simulink model "dec_fir_dbl_col_test"  (Simulink 7.2)
settings: Solver=FixedStepDiscrete  SolverMode=SingleTasking  StartTime=0.0  StopTime=50  RelTol=1e-3
libraries: xbsIndex_r4 x50, casper_library_downconverter x8, casper_library_misc x2
settings Model: Creator=User  LastModifiedBy=root
settings OptimizationCC: InitFltsAndDblsToZero=on

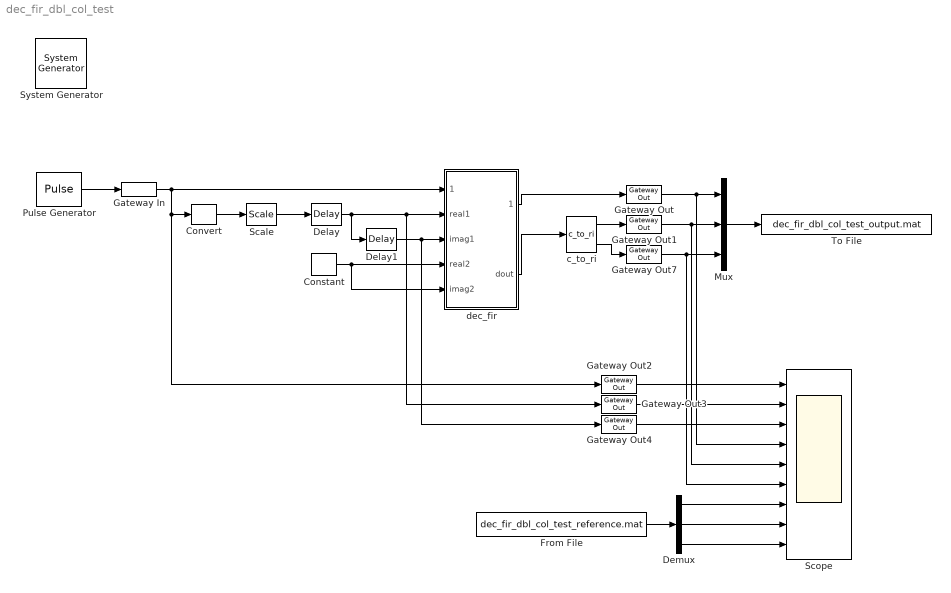
== system dec_fir_dbl_col_test ==
  " System Generator" : xbsIndex_r4/ System Generator  Tag=genX  SystemSampleTime=-1  xilinxfamily=Virtex4  part=xc4vsx35  speed=-10  package=ff668  synthesis_tool=XST  clock_wrapper=Clock Enables  directory=./netlist  testbench=off  simulink_period=1  sysclk_period=100  dcm_input_clock_period=100  incr_netlist=off  trim_vbits=Everywhere in SubSystem  dbl_ovrd=According to Block Masks  core_generation=According to Block Masks  run_coregen=off  deprecated_control=off  eval_field=0  block_type=sysgen
      settings: block_version=10.1.1
  Constant : xbsIndex_r4/Constant  arith_type=Signed (2's comp)  const=0  n_bits=10  bin_pt=9  explicit_period=on  period=1  equ=P=C  opselect=C  inp2=PCIN>>17  opr=+  inp1=P  carry=CIN  dbl_ovrd=off  block_type=constant
      settings: block_version=11.4
  Convert : xbsIndex_r4/Convert  arith_type="Signed  (2's comp)"  n_bits=10  bin_pt=8  quantization=Truncate  overflow=Wrap  latency=0  dbl_ovrd=off  pipeline=off  block_type=convert
      settings: block_version=11.4
  Delay : xbsIndex_r4/Delay  en=off  latency=1  dbl_ovrd=off  reg_retiming=off  block_type=delay
      settings: block_version=11.4
  Delay1 : xbsIndex_r4/Delay  en=off  latency=1  dbl_ovrd=off  reg_retiming=off  block_type=delay
      settings: block_version=11.4
  Demux : Demux  Outputs=3
  From File : FromFile  FileName=dec_fir_dbl_col_test_reference.mat  SampleTime=1
  Gateway In : xbsIndex_r4/Gateway In  arith_type=Boolean  n_bits=16  bin_pt=14  quantization="Round  (unbiased: +/- Inf)"  overflow=Saturate  period=1  dbl_ovrd=off  timing_constraint=None  locs_specified=off  LOCs={}  hdl_port=on  block_type=gatewayin
      settings: infoedit="Gateway in block.  Converts inputs of type Simulink integer, double and fixed point to  Xilinx fixed point type.<P><P>Hardware notes:  In hardware these blocks become top level input ports."  block_version=10.1.1
  Gateway Out{,1..4,7} (6 alike) : xbsIndex_r4/Gateway Out  hdl_port=on  timing_constraint=None  locs_specified=off  LOCs={}  block_type=gatewayout
      settings: infoedit="Gateway out block.  Converts Xilinx fixed point inputs into ouputs of type Simulink integer, double, or fixed point.<br><br>Hardware notes:  In hardware these blocks become top level output ports or are discarded, depending on how they are configured."  block_version=11.4
  Mux : Mux  Inputs=3
  Pulse Generator : DiscretePulseGenerator  Period=128  PhaseDelay=15
  Scale : xbsIndex_r4/Scale  scale_factor=-1  dbl_ovrd=off  block_type=scale
  Scope : Scope  NumInputPorts=9
      settings: YMin=-5~-5~-5~-5~-5~-5~-5~-5~-5  YMax=5~5~5~5~5~5~5~5~5
  To File : ToFile  Filename=dec_fir_dbl_col_test_output.mat  MatrixName=output
  c_to_ri : casper_library_misc/c_to_ri  SystemSampleTime=-1  n_bits=10  bin_pt=9
      settings: AttributesFormatString=10_9 r/i
  dec_fir : Subsystem  AncestorBlock=casper_library_downconverter/dec_fir  mask(dec_fir){n_inputs=2, coeff=getfield( getfield( get_param( gcb,'UserData' ), 'parameters'),'coeff'), n_bits=10, quantization=Round  (unbiased: Even Values), add_latency=2, mult_latency=3, conv_latency=2, coeff_bit_width=18, coeff_bin_pt=17, absorb_adders=off, adder_imp=DSP48}
      mask prompts: n_inputs "Number of Parallel Streams"; coeff "Coefficients"; n_bits "Bit Width Out"; quantization "Quantization Behavior"; add_latency "Add Latency"; mult_latency "Mult Latency"; conv_latency "Convert latency"; coeff_bit_width "Coefficient bit width"; coeff_bin_pt "Coefficient binary point"; absorb_adders "Absorb adders into DSP slices"; adder_imp "Adder implementation"
      mask help: FIR filter which can handle multiple time samples in parallel and decimates down to 1 time sample. If coefficients are symmetric, will automatically fold before multiplying.
      mask init:
      | dec_fir_init(gcb, ...
      |     'n_inputs', n_inputs, ...
      |     'coeff', coeff, ...
      |     'n_bits', n_bits, ...
      |     'quantization', quantization, ...
      |     'add_latency', add_latency, ...
      |     'mult_latency', mult_latency, ...
      |     'conv_latency', conv_latency, ...
      |     'coeff_bit_width', coeff_bit_width, ...
      |     'coeff_bin_pt', coeff_bin_pt, ...
      |     'absorb_adders', absorb_adders, ...
      |     'adder_imp', adder_imp);
      settings: AttributesFormatString=|
      | 16 taps
      | 10_9 r/i
      mask Help: eval('xlWeb(''http://casper.berkeley.edu/wiki/Dec_fir'')')
      mask StyleString: edit,edit,edit,popup(Truncate|Round  (unbiased: +/- Inf)|Round  (unbiased: Even Values)),edit,edit,edit,edit,edit,checkbox,popup(Behavioral|Fabric|DSP48)
  wires:
  Pulse Generator/1 -> Gateway In/1
  Gateway In/1 -> Convert/1, Gateway Out2/1, dec_fir/1(sync_in)
  Mux/1 -> To File/1
  Delay/1 -> Delay1/1, Gateway Out3/1, dec_fir/2(real1)
  Delay1/1 -> Gateway Out4/1, dec_fir/3(imag1)
  Convert/1 -> Scale/1
  Gateway Out/1 -> Mux/1, Scope/4
  Gateway Out2/1 -> Scope/1
  Gateway Out3/1 -> Scope/2
  Gateway Out4/1 -> Scope/3
  dec_fir/2(dout) -> c_to_ri/1
  c_to_ri/1 -> Gateway Out1/1
  c_to_ri/2 -> Gateway Out7/1
  Gateway Out1/1 -> Mux/2, Scope/5
  From File/1 -> Demux/1
  Scale/1 -> Delay/1
  dec_fir/1(sync_out) -> Gateway Out/1
  Gateway Out7/1 -> Mux/3, Scope/6
  Demux/1 -> Scope/7
  Demux/2 -> Scope/8
  Demux/3 -> Scope/9
  Constant/1 -> dec_fir/5(imag2), dec_fir/4(real2)

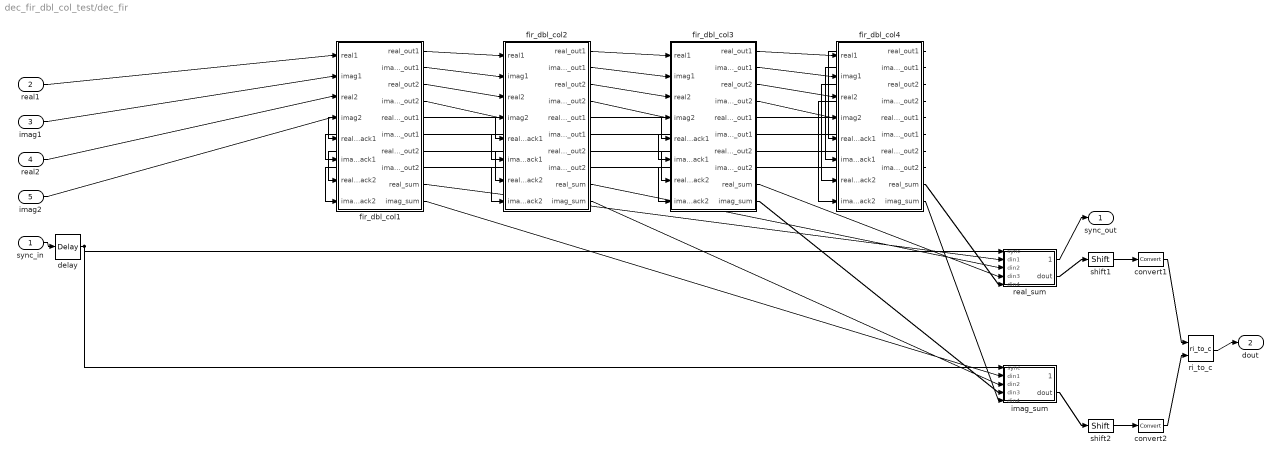
== system dec_fir_dbl_col_test/dec_fir ==
  sync_in : Inport
  real1 : Inport  Port=2
  imag1 : Inport  Port=3
  real2 : Inport  Port=4
  imag2 : Inport  Port=5
  convert1 : xbsIndex_r4/Convert  arith_type="Signed  (2's comp)"  n_bits=10  bin_pt=9  quantization="Round  (unbiased: Even Values)"  overflow=Wrap  latency=2  dbl_ovrd=off  pipeline=off  block_type=convert
      settings: block_version=11.4
  convert2 : xbsIndex_r4/Convert  arith_type="Signed  (2's comp)"  n_bits=10  bin_pt=9  quantization="Round  (unbiased: Even Values)"  overflow=Wrap  latency=2  dbl_ovrd=off  pipeline=off  block_type=convert
      settings: block_version=11.4
  delay : xbsIndex_r4/Delay  en=off  latency=9  dbl_ovrd=off  reg_retiming=off  block_type=delay
      settings: block_version=11.4
  fir_dbl_col1 : Subsystem  AncestorBlock=casper_library_downconverter/fir_dbl_col  mask(fir_dbl_col){n_inputs=2, coeff=[0.2         0.1], add_latency=2, mult_latency=3, coeff_bit_width=18, coeff_bin_pt=17, first_stage_hdl=off, adder_imp=DSP48}
      mask prompts: n_inputs "Inputs"; coeff "Coefficients"; add_latency "Add latency"; mult_latency "Mult Latency"; coeff_bit_width "Coefficient bit width"; coeff_bin_pt "Coefficient binary point"; first_stage_hdl "Implement first stage of adder trees on output as behavioural HDL"; adder_imp "Adder implementation"
      mask init:
      | fir_dbl_col_init(gcb, ...
      |     'n_inputs', n_inputs, ...
      |     'coeff', coeff, ...
      |     'mult_latency', mult_latency, ...
      |     'add_latency', add_latency, ...
      |     'coeff_bit_width', coeff_bit_width, ...
      |     'coeff_bin_pt', coeff_bin_pt,  ...
      |     'first_stage_hdl', first_stage_hdl, ...
      |     'adder_imp', adder_imp);
      mask Help: eval('xlWeb(''http://casper.berkeley.edu/wiki/Fir_dbl_col'')')
      mask StyleString: edit,edit,edit,edit,edit,edit,checkbox,popup(Behavioral|Fabric|DSP48)
  fir_dbl_col2 : Subsystem  AncestorBlock=casper_library_downconverter/fir_dbl_col  mask(fir_dbl_col){n_inputs=2, coeff=[0.4         0.3], add_latency=2, mult_latency=3, coeff_bit_width=18, coeff_bin_pt=17, first_stage_hdl=off, adder_imp=DSP48}
      mask prompts: n_inputs "Inputs"; coeff "Coefficients"; add_latency "Add latency"; mult_latency "Mult Latency"; coeff_bit_width "Coefficient bit width"; coeff_bin_pt "Coefficient binary point"; first_stage_hdl "Implement first stage of adder trees on output as behavioural HDL"; adder_imp "Adder implementation"
      mask init: same as dec_fir_dbl_col_test/dec_fir/fir_dbl_col1
      mask Help: eval('xlWeb(''http://casper.berkeley.edu/wiki/Fir_dbl_col'')')
      mask StyleString: edit,edit,edit,edit,edit,edit,checkbox,popup(Behavioral|Fabric|DSP48)
  fir_dbl_col3 : Subsystem  AncestorBlock=casper_library_downconverter/fir_dbl_col  mask(fir_dbl_col){n_inputs=2, coeff=[0.6         0.5], add_latency=2, mult_latency=3, coeff_bit_width=18, coeff_bin_pt=17, first_stage_hdl=off, adder_imp=DSP48}
      mask prompts: n_inputs "Inputs"; coeff "Coefficients"; add_latency "Add latency"; mult_latency "Mult Latency"; coeff_bit_width "Coefficient bit width"; coeff_bin_pt "Coefficient binary point"; first_stage_hdl "Implement first stage of adder trees on output as behavioural HDL"; adder_imp "Adder implementation"
      mask init: same as dec_fir_dbl_col_test/dec_fir/fir_dbl_col1
      mask Help: eval('xlWeb(''http://casper.berkeley.edu/wiki/Fir_dbl_col'')')
      mask StyleString: edit,edit,edit,edit,edit,edit,checkbox,popup(Behavioral|Fabric|DSP48)
  fir_dbl_col4 : Subsystem  AncestorBlock=casper_library_downconverter/fir_dbl_col  mask(fir_dbl_col){n_inputs=2, coeff=[0.8         0.7], add_latency=2, mult_latency=3, coeff_bit_width=18, coeff_bin_pt=17, first_stage_hdl=off, adder_imp=DSP48}
      mask prompts: n_inputs "Inputs"; coeff "Coefficients"; add_latency "Add latency"; mult_latency "Mult Latency"; coeff_bit_width "Coefficient bit width"; coeff_bin_pt "Coefficient binary point"; first_stage_hdl "Implement first stage of adder trees on output as behavioural HDL"; adder_imp "Adder implementation"
      mask init: same as dec_fir_dbl_col_test/dec_fir/fir_dbl_col1
      mask Help: eval('xlWeb(''http://casper.berkeley.edu/wiki/Fir_dbl_col'')')
      mask StyleString: edit,edit,edit,edit,edit,edit,checkbox,popup(Behavioral|Fabric|DSP48)
  imag_sum : Subsystem  AncestorBlock=casper_library_misc/adder_tree  mask(adder_tree){n_inputs=4, latency=2, adder_imp=DSP48, first_stage_hdl=off}
      mask prompts: n_inputs "Number of Inputs"; latency "Add Latency"; adder_imp "Adder implementation"; first_stage_hdl "Use behavioural HDL for first stage of adders"
      mask help:
      | Sums all inputs using a tree of adds and delays.
      |
      | Number of inputs: The number of inputs to the block to be summed
      | Add latency: The number of clock cycles to perform one addition (affects timing)..
      | Adder implementation: choice of fabric or DSP48E core, or behavioral HDL
      | Use behavioural HDL for first stage of adders: Causes the first stage of adders to be absorbed into DSP blocks if multipliers precede them (Virtex 5). Overrides Adder implementation
      mask init:
      | adder_tree_init(gcb, ...
      |     'n_inputs', n_inputs, ...
      |     'latency', latency, ...
      |     'adder_imp', adder_imp, ...
      |     'first_stage_hdl', first_stage_hdl);
      settings: AttributesFormatString=latency 4
      mask Help: eval('xlWeb(''http://casper.berkeley.edu/wiki/Adder_tree'')')
      mask StyleString: edit,edit,popup(Behavioral|Fabric|DSP48),checkbox
  real_sum : Subsystem  AncestorBlock=casper_library_misc/adder_tree  mask(adder_tree){n_inputs=4, latency=2, adder_imp=DSP48, first_stage_hdl=off}
      mask prompts: n_inputs "Number of Inputs"; latency "Add Latency"; adder_imp "Adder implementation"; first_stage_hdl "Use behavioural HDL for first stage of adders"
      mask help:
      | Sums all inputs using a tree of adds and delays.
      |
      | Number of inputs: The number of inputs to the block to be summed
      | Add latency: The number of clock cycles to perform one addition (affects timing)..
      | Adder implementation: choice of fabric or DSP48E core, or behavioral HDL
      | Use behavioural HDL for first stage of adders: Causes the first stage of adders to be absorbed into DSP blocks if multipliers precede them (Virtex 5). Overrides Adder implementation
      mask init:
      | adder_tree_init(gcb, ...
      |     'n_inputs', n_inputs, ...
      |     'latency', latency, ...
      |     'adder_imp', adder_imp, ...
      |     'first_stage_hdl', first_stage_hdl);
      settings: AttributesFormatString=latency 4
      mask Help: eval('xlWeb(''http://casper.berkeley.edu/wiki/Adder_tree'')')
      mask StyleString: edit,edit,popup(Behavioral|Fabric|DSP48),checkbox
  ri_to_c : casper_library_misc/ri_to_c  SystemSampleTime=-1
  shift1 : xbsIndex_r4/Shift  shift_dir=Left  shift_bits=1  en=off  latency=0  precision=Full  arith_type="Signed  (2's comp)"  n_bits=16  bin_pt=14  quantization=Truncate  overflow=Wrap  dbl_ovrd=off  block_type=shift
  shift2 : xbsIndex_r4/Shift  shift_dir=Left  shift_bits=1  en=off  latency=0  precision=Full  arith_type="Signed  (2's comp)"  n_bits=16  bin_pt=14  quantization=Truncate  overflow=Wrap  dbl_ovrd=off  block_type=shift
  sync_out : Outport
  dout : Outport  Port=2
  wires:
  real1/1 -> fir_dbl_col1/1(real1)
  imag1/1 -> fir_dbl_col1/2(imag1)
  real2/1 -> fir_dbl_col1/3(real2)
  imag2/1 -> fir_dbl_col1/4(imag2)
  fir_dbl_col1/9(real_sum) -> real_sum/2(din1)
  fir_dbl_col1/10(imag_sum) -> imag_sum/2(din1)
  fir_dbl_col1/1(real_out1) -> fir_dbl_col2/1(real1)
  fir_dbl_col1/2(imag_out1) -> fir_dbl_col2/2(imag1)
  fir_dbl_col1/3(real_out2) -> fir_dbl_col2/3(real2)
  fir_dbl_col1/4(imag_out2) -> fir_dbl_col2/4(imag2)
  fir_dbl_col2/9(real_sum) -> real_sum/3(din2)
  fir_dbl_col2/10(imag_sum) -> imag_sum/3(din2)
  fir_dbl_col2/1(real_out1) -> fir_dbl_col3/1(real1)
  fir_dbl_col2/2(imag_out1) -> fir_dbl_col3/2(imag1)
  fir_dbl_col2/3(real_out2) -> fir_dbl_col3/3(real2)
  fir_dbl_col2/4(imag_out2) -> fir_dbl_col3/4(imag2)
  fir_dbl_col3/9(real_sum) -> real_sum/4(din3)
  fir_dbl_col3/10(imag_sum) -> imag_sum/4(din3)
  fir_dbl_col3/1(real_out1) -> fir_dbl_col4/1(real1)
  fir_dbl_col3/2(imag_out1) -> fir_dbl_col4/2(imag1)
  fir_dbl_col3/3(real_out2) -> fir_dbl_col4/3(real2)
  fir_dbl_col3/4(imag_out2) -> fir_dbl_col4/4(imag2)
  fir_dbl_col4/9(real_sum) -> real_sum/5(din4)
  fir_dbl_col4/10(imag_sum) -> imag_sum/5(din4)
  real_sum/2(dout) -> shift1/1
  imag_sum/2(dout) -> shift2/1
  shift1/1 -> convert1/1
  shift2/1 -> convert2/1
  convert1/1 -> ri_to_c/1
  convert2/1 -> ri_to_c/2
  ri_to_c/1 -> dout/1
  sync_in/1 -> delay/1
  delay/1 -> real_sum/1(sync), imag_sum/1(sync)
  real_sum/1(sync_out) -> sync_out/1
  fir_dbl_col2/5(real_back_out1) -> fir_dbl_col1/5(real_back1)
  fir_dbl_col2/6(imag_back_out1) -> fir_dbl_col1/6(imag_back1)
  fir_dbl_col2/7(real_back_out2) -> fir_dbl_col1/7(real_back2)
  fir_dbl_col2/8(imag_back_out2) -> fir_dbl_col1/8(imag_back2)
  fir_dbl_col3/5(real_back_out1) -> fir_dbl_col2/5(real_back1)
  fir_dbl_col3/6(imag_back_out1) -> fir_dbl_col2/6(imag_back1)
  fir_dbl_col3/7(real_back_out2) -> fir_dbl_col2/7(real_back2)
  fir_dbl_col3/8(imag_back_out2) -> fir_dbl_col2/8(imag_back2)
  fir_dbl_col4/5(real_back_out1) -> fir_dbl_col3/5(real_back1)
  fir_dbl_col4/6(imag_back_out1) -> fir_dbl_col3/6(imag_back1)
  fir_dbl_col4/7(real_back_out2) -> fir_dbl_col3/7(real_back2)
  fir_dbl_col4/8(imag_back_out2) -> fir_dbl_col3/8(imag_back2)
  fir_dbl_col4/1(real_out1) -> fir_dbl_col4/5(real_back1)
  fir_dbl_col4/2(imag_out1) -> fir_dbl_col4/6(imag_back1)
  fir_dbl_col4/3(real_out2) -> fir_dbl_col4/7(real_back2)
  fir_dbl_col4/4(imag_out2) -> fir_dbl_col4/8(imag_back2)

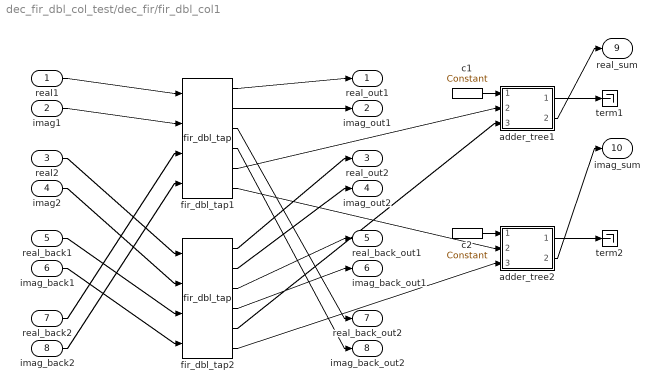
== system dec_fir_dbl_col_test/dec_fir/fir_dbl_col1 ==
  real1 : Inport
  imag1 : Inport  Port=2
  real2 : Inport  Port=3
  imag2 : Inport  Port=4
  real_back1 : Inport  Port=5
  imag_back1 : Inport  Port=6
  real_back2 : Inport  Port=7
  imag_back2 : Inport  Port=8
  adder_tree1 : Subsystem  AncestorBlock=casper_library_misc/adder_tree  mask(adder_tree){n_inputs=2, latency=2, adder_imp=DSP48, first_stage_hdl=off}
      mask prompts: n_inputs "Number of Inputs"; latency "Add Latency"; adder_imp "Adder implementation"; first_stage_hdl "Use behavioural HDL for first stage of adders"
      mask help:
      | Sums all inputs using a tree of adds and delays.
      |
      | Number of inputs: The number of inputs to the block to be summed
      | Add latency: The number of clock cycles to perform one addition (affects timing)..
      | Adder implementation: choice of fabric or DSP48E core, or behavioral HDL
      | Use behavioural HDL for first stage of adders: Causes the first stage of adders to be absorbed into DSP blocks if multipliers precede them (Virtex 5). Overrides Adder implementation
      mask init:
      | adder_tree_init(gcb, ...
      |     'n_inputs', n_inputs, ...
      |     'latency', latency, ...
      |     'adder_imp', adder_imp, ...
      |     'first_stage_hdl', first_stage_hdl);
      settings: AttributesFormatString=latency 2
      mask Help: eval('xlWeb(''http://casper.berkeley.edu/wiki/Adder_tree'')')
      mask StyleString: edit,edit,popup(Behavioral|Fabric|DSP48),checkbox
  adder_tree2 : Subsystem  AncestorBlock=casper_library_misc/adder_tree  mask(adder_tree){n_inputs=2, latency=2, adder_imp=DSP48, first_stage_hdl=off}
      mask prompts: n_inputs "Number of Inputs"; latency "Add Latency"; adder_imp "Adder implementation"; first_stage_hdl "Use behavioural HDL for first stage of adders"
      mask help:
      | Sums all inputs using a tree of adds and delays.
      |
      | Number of inputs: The number of inputs to the block to be summed
      | Add latency: The number of clock cycles to perform one addition (affects timing)..
      | Adder implementation: choice of fabric or DSP48E core, or behavioral HDL
      | Use behavioural HDL for first stage of adders: Causes the first stage of adders to be absorbed into DSP blocks if multipliers precede them (Virtex 5). Overrides Adder implementation
      mask init:
      | adder_tree_init(gcb, ...
      |     'n_inputs', n_inputs, ...
      |     'latency', latency, ...
      |     'adder_imp', adder_imp, ...
      |     'first_stage_hdl', first_stage_hdl);
      settings: AttributesFormatString=latency 2
      mask Help: eval('xlWeb(''http://casper.berkeley.edu/wiki/Adder_tree'')')
      mask StyleString: edit,edit,popup(Behavioral|Fabric|DSP48),checkbox
  c1 : xbsIndex_r4/Constant  arith_type=Signed (2's comp)  const=1  n_bits=16  bin_pt=14  explicit_period=on  period=1  equ=P=C  opselect=C  inp2=PCIN>>17  opr=+  inp1=P  carry=CIN  dbl_ovrd=off  block_type=constant
      settings: block_version=11.4
  c2 : xbsIndex_r4/Constant  arith_type=Signed (2's comp)  const=1  n_bits=16  bin_pt=14  explicit_period=on  period=1  equ=P=C  opselect=C  inp2=PCIN>>17  opr=+  inp1=P  carry=CIN  dbl_ovrd=off  block_type=constant
      settings: block_version=11.4
  fir_dbl_tap1 : casper_library_downconverter/fir_dbl_tap  SystemSampleTime=-1  factor=0.2  add_latency=2  mult_latency=3  coeff_bit_width=18  coeff_bin_pt=17
  fir_dbl_tap2 : casper_library_downconverter/fir_dbl_tap  SystemSampleTime=-1  factor=0.1  add_latency=2  mult_latency=3  coeff_bit_width=18  coeff_bin_pt=17
  term1 : Terminator
  term2 : Terminator
  real_out1 : Outport
  imag_out1 : Outport  Port=2
  real_out2 : Outport  Port=3
  imag_out2 : Outport  Port=4
  real_back_out1 : Outport  Port=5
  imag_back_out1 : Outport  Port=6
  real_back_out2 : Outport  Port=7
  imag_back_out2 : Outport  Port=8
  real_sum : Outport  Port=9
  imag_sum : Outport  Port=10
  wires:
  adder_tree1/1(sync_out) -> term1/1
  adder_tree2/1(sync_out) -> term2/1
  c1/1 -> adder_tree1/1(sync)
  c2/1 -> adder_tree2/1(sync)
  adder_tree1/2(dout) -> real_sum/1
  adder_tree2/2(dout) -> imag_sum/1
  real1/1 -> fir_dbl_tap1/1
  imag1/1 -> fir_dbl_tap1/2
  real_back2/1 -> fir_dbl_tap1/3
  imag_back2/1 -> fir_dbl_tap1/4
  fir_dbl_tap1/1 -> real_out1/1
  fir_dbl_tap1/2 -> imag_out1/1
  fir_dbl_tap1/3 -> real_back_out2/1
  fir_dbl_tap1/4 -> imag_back_out2/1
  fir_dbl_tap1/5 -> adder_tree1/2(din1)
  fir_dbl_tap1/6 -> adder_tree2/2(din1)
  real2/1 -> fir_dbl_tap2/1
  imag2/1 -> fir_dbl_tap2/2
  real_back1/1 -> fir_dbl_tap2/3
  imag_back1/1 -> fir_dbl_tap2/4
  fir_dbl_tap2/1 -> real_out2/1
  fir_dbl_tap2/2 -> imag_out2/1
  fir_dbl_tap2/3 -> real_back_out1/1
  fir_dbl_tap2/4 -> imag_back_out1/1
  fir_dbl_tap2/5 -> adder_tree1/3(din2)
  fir_dbl_tap2/6 -> adder_tree2/3(din2)

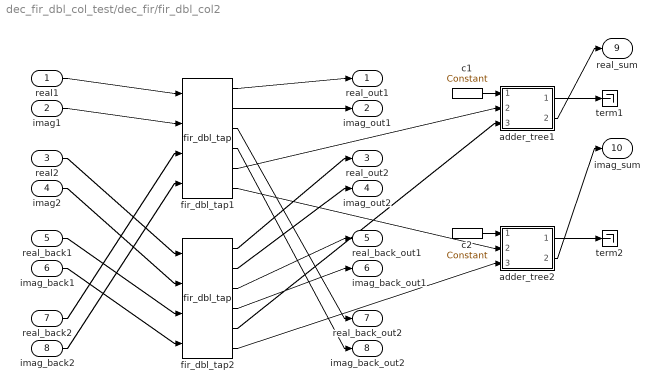
== system dec_fir_dbl_col_test/dec_fir/fir_dbl_col2 ==
  real1 : Inport
  imag1 : Inport  Port=2
  real2 : Inport  Port=3
  imag2 : Inport  Port=4
  real_back1 : Inport  Port=5
  imag_back1 : Inport  Port=6
  real_back2 : Inport  Port=7
  imag_back2 : Inport  Port=8
  adder_tree1 : Subsystem  AncestorBlock=casper_library_misc/adder_tree  mask(adder_tree){n_inputs=2, latency=2, adder_imp=DSP48, first_stage_hdl=off}
      mask prompts: n_inputs "Number of Inputs"; latency "Add Latency"; adder_imp "Adder implementation"; first_stage_hdl "Use behavioural HDL for first stage of adders"
      mask help:
      | Sums all inputs using a tree of adds and delays.
      |
      | Number of inputs: The number of inputs to the block to be summed
      | Add latency: The number of clock cycles to perform one addition (affects timing)..
      | Adder implementation: choice of fabric or DSP48E core, or behavioral HDL
      | Use behavioural HDL for first stage of adders: Causes the first stage of adders to be absorbed into DSP blocks if multipliers precede them (Virtex 5). Overrides Adder implementation
      mask init:
      | adder_tree_init(gcb, ...
      |     'n_inputs', n_inputs, ...
      |     'latency', latency, ...
      |     'adder_imp', adder_imp, ...
      |     'first_stage_hdl', first_stage_hdl);
      settings: AttributesFormatString=latency 2
      mask Help: eval('xlWeb(''http://casper.berkeley.edu/wiki/Adder_tree'')')
      mask StyleString: edit,edit,popup(Behavioral|Fabric|DSP48),checkbox
  adder_tree2 : Subsystem  AncestorBlock=casper_library_misc/adder_tree  mask(adder_tree){n_inputs=2, latency=2, adder_imp=DSP48, first_stage_hdl=off}
      mask prompts: n_inputs "Number of Inputs"; latency "Add Latency"; adder_imp "Adder implementation"; first_stage_hdl "Use behavioural HDL for first stage of adders"
      mask help:
      | Sums all inputs using a tree of adds and delays.
      |
      | Number of inputs: The number of inputs to the block to be summed
      | Add latency: The number of clock cycles to perform one addition (affects timing)..
      | Adder implementation: choice of fabric or DSP48E core, or behavioral HDL
      | Use behavioural HDL for first stage of adders: Causes the first stage of adders to be absorbed into DSP blocks if multipliers precede them (Virtex 5). Overrides Adder implementation
      mask init:
      | adder_tree_init(gcb, ...
      |     'n_inputs', n_inputs, ...
      |     'latency', latency, ...
      |     'adder_imp', adder_imp, ...
      |     'first_stage_hdl', first_stage_hdl);
      settings: AttributesFormatString=latency 2
      mask Help: eval('xlWeb(''http://casper.berkeley.edu/wiki/Adder_tree'')')
      mask StyleString: edit,edit,popup(Behavioral|Fabric|DSP48),checkbox
  c1 : xbsIndex_r4/Constant  arith_type=Signed (2's comp)  const=1  n_bits=16  bin_pt=14  explicit_period=on  period=1  equ=P=C  opselect=C  inp2=PCIN>>17  opr=+  inp1=P  carry=CIN  dbl_ovrd=off  block_type=constant
      settings: block_version=11.4
  c2 : xbsIndex_r4/Constant  arith_type=Signed (2's comp)  const=1  n_bits=16  bin_pt=14  explicit_period=on  period=1  equ=P=C  opselect=C  inp2=PCIN>>17  opr=+  inp1=P  carry=CIN  dbl_ovrd=off  block_type=constant
      settings: block_version=11.4
  fir_dbl_tap1 : casper_library_downconverter/fir_dbl_tap  SystemSampleTime=-1  factor=0.4  add_latency=2  mult_latency=3  coeff_bit_width=18  coeff_bin_pt=17
  fir_dbl_tap2 : casper_library_downconverter/fir_dbl_tap  SystemSampleTime=-1  factor=0.3  add_latency=2  mult_latency=3  coeff_bit_width=18  coeff_bin_pt=17
  term1 : Terminator
  term2 : Terminator
  real_out1 : Outport
  imag_out1 : Outport  Port=2
  real_out2 : Outport  Port=3
  imag_out2 : Outport  Port=4
  real_back_out1 : Outport  Port=5
  imag_back_out1 : Outport  Port=6
  real_back_out2 : Outport  Port=7
  imag_back_out2 : Outport  Port=8
  real_sum : Outport  Port=9
  imag_sum : Outport  Port=10
  wires:
  adder_tree1/1(sync_out) -> term1/1
  adder_tree2/1(sync_out) -> term2/1
  c1/1 -> adder_tree1/1(sync)
  c2/1 -> adder_tree2/1(sync)
  adder_tree1/2(dout) -> real_sum/1
  adder_tree2/2(dout) -> imag_sum/1
  real1/1 -> fir_dbl_tap1/1
  imag1/1 -> fir_dbl_tap1/2
  real_back2/1 -> fir_dbl_tap1/3
  imag_back2/1 -> fir_dbl_tap1/4
  fir_dbl_tap1/1 -> real_out1/1
  fir_dbl_tap1/2 -> imag_out1/1
  fir_dbl_tap1/3 -> real_back_out2/1
  fir_dbl_tap1/4 -> imag_back_out2/1
  fir_dbl_tap1/5 -> adder_tree1/2(din1)
  fir_dbl_tap1/6 -> adder_tree2/2(din1)
  real2/1 -> fir_dbl_tap2/1
  imag2/1 -> fir_dbl_tap2/2
  real_back1/1 -> fir_dbl_tap2/3
  imag_back1/1 -> fir_dbl_tap2/4
  fir_dbl_tap2/1 -> real_out2/1
  fir_dbl_tap2/2 -> imag_out2/1
  fir_dbl_tap2/3 -> real_back_out1/1
  fir_dbl_tap2/4 -> imag_back_out1/1
  fir_dbl_tap2/5 -> adder_tree1/3(din2)
  fir_dbl_tap2/6 -> adder_tree2/3(din2)

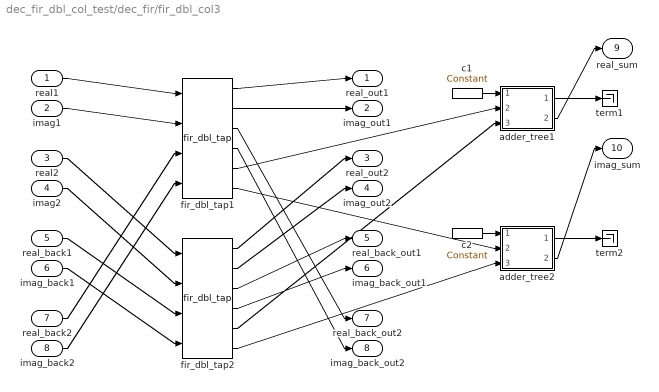
== system dec_fir_dbl_col_test/dec_fir/fir_dbl_col3 ==
  real1 : Inport
  imag1 : Inport  Port=2
  real2 : Inport  Port=3
  imag2 : Inport  Port=4
  real_back1 : Inport  Port=5
  imag_back1 : Inport  Port=6
  real_back2 : Inport  Port=7
  imag_back2 : Inport  Port=8
  adder_tree1 : Subsystem  AncestorBlock=casper_library_misc/adder_tree  mask(adder_tree){n_inputs=2, latency=2, adder_imp=DSP48, first_stage_hdl=off}
      mask prompts: n_inputs "Number of Inputs"; latency "Add Latency"; adder_imp "Adder implementation"; first_stage_hdl "Use behavioural HDL for first stage of adders"
      mask help:
      | Sums all inputs using a tree of adds and delays.
      |
      | Number of inputs: The number of inputs to the block to be summed
      | Add latency: The number of clock cycles to perform one addition (affects timing)..
      | Adder implementation: choice of fabric or DSP48E core, or behavioral HDL
      | Use behavioural HDL for first stage of adders: Causes the first stage of adders to be absorbed into DSP blocks if multipliers precede them (Virtex 5). Overrides Adder implementation
      mask init:
      | adder_tree_init(gcb, ...
      |     'n_inputs', n_inputs, ...
      |     'latency', latency, ...
      |     'adder_imp', adder_imp, ...
      |     'first_stage_hdl', first_stage_hdl);
      settings: AttributesFormatString=latency 2
      mask Help: eval('xlWeb(''http://casper.berkeley.edu/wiki/Adder_tree'')')
      mask StyleString: edit,edit,popup(Behavioral|Fabric|DSP48),checkbox
  adder_tree2 : Subsystem  AncestorBlock=casper_library_misc/adder_tree  mask(adder_tree){n_inputs=2, latency=2, adder_imp=DSP48, first_stage_hdl=off}
      mask prompts: n_inputs "Number of Inputs"; latency "Add Latency"; adder_imp "Adder implementation"; first_stage_hdl "Use behavioural HDL for first stage of adders"
      mask help:
      | Sums all inputs using a tree of adds and delays.
      |
      | Number of inputs: The number of inputs to the block to be summed
      | Add latency: The number of clock cycles to perform one addition (affects timing)..
      | Adder implementation: choice of fabric or DSP48E core, or behavioral HDL
      | Use behavioural HDL for first stage of adders: Causes the first stage of adders to be absorbed into DSP blocks if multipliers precede them (Virtex 5). Overrides Adder implementation
      mask init:
      | adder_tree_init(gcb, ...
      |     'n_inputs', n_inputs, ...
      |     'latency', latency, ...
      |     'adder_imp', adder_imp, ...
      |     'first_stage_hdl', first_stage_hdl);
      settings: AttributesFormatString=latency 2
      mask Help: eval('xlWeb(''http://casper.berkeley.edu/wiki/Adder_tree'')')
      mask StyleString: edit,edit,popup(Behavioral|Fabric|DSP48),checkbox
  c1 : xbsIndex_r4/Constant  arith_type=Signed (2's comp)  const=1  n_bits=16  bin_pt=14  explicit_period=on  period=1  equ=P=C  opselect=C  inp2=PCIN>>17  opr=+  inp1=P  carry=CIN  dbl_ovrd=off  block_type=constant
      settings: block_version=11.4
  c2 : xbsIndex_r4/Constant  arith_type=Signed (2's comp)  const=1  n_bits=16  bin_pt=14  explicit_period=on  period=1  equ=P=C  opselect=C  inp2=PCIN>>17  opr=+  inp1=P  carry=CIN  dbl_ovrd=off  block_type=constant
      settings: block_version=11.4
  fir_dbl_tap1 : casper_library_downconverter/fir_dbl_tap  SystemSampleTime=-1  factor=0.6  add_latency=2  mult_latency=3  coeff_bit_width=18  coeff_bin_pt=17
  fir_dbl_tap2 : casper_library_downconverter/fir_dbl_tap  SystemSampleTime=-1  factor=0.5  add_latency=2  mult_latency=3  coeff_bit_width=18  coeff_bin_pt=17
  term1 : Terminator
  term2 : Terminator
  real_out1 : Outport
  imag_out1 : Outport  Port=2
  real_out2 : Outport  Port=3
  imag_out2 : Outport  Port=4
  real_back_out1 : Outport  Port=5
  imag_back_out1 : Outport  Port=6
  real_back_out2 : Outport  Port=7
  imag_back_out2 : Outport  Port=8
  real_sum : Outport  Port=9
  imag_sum : Outport  Port=10
  wires:
  adder_tree1/1(sync_out) -> term1/1
  adder_tree2/1(sync_out) -> term2/1
  c1/1 -> adder_tree1/1(sync)
  c2/1 -> adder_tree2/1(sync)
  adder_tree1/2(dout) -> real_sum/1
  adder_tree2/2(dout) -> imag_sum/1
  real1/1 -> fir_dbl_tap1/1
  imag1/1 -> fir_dbl_tap1/2
  real_back2/1 -> fir_dbl_tap1/3
  imag_back2/1 -> fir_dbl_tap1/4
  fir_dbl_tap1/1 -> real_out1/1
  fir_dbl_tap1/2 -> imag_out1/1
  fir_dbl_tap1/3 -> real_back_out2/1
  fir_dbl_tap1/4 -> imag_back_out2/1
  fir_dbl_tap1/5 -> adder_tree1/2(din1)
  fir_dbl_tap1/6 -> adder_tree2/2(din1)
  real2/1 -> fir_dbl_tap2/1
  imag2/1 -> fir_dbl_tap2/2
  real_back1/1 -> fir_dbl_tap2/3
  imag_back1/1 -> fir_dbl_tap2/4
  fir_dbl_tap2/1 -> real_out2/1
  fir_dbl_tap2/2 -> imag_out2/1
  fir_dbl_tap2/3 -> real_back_out1/1
  fir_dbl_tap2/4 -> imag_back_out1/1
  fir_dbl_tap2/5 -> adder_tree1/3(din2)
  fir_dbl_tap2/6 -> adder_tree2/3(din2)

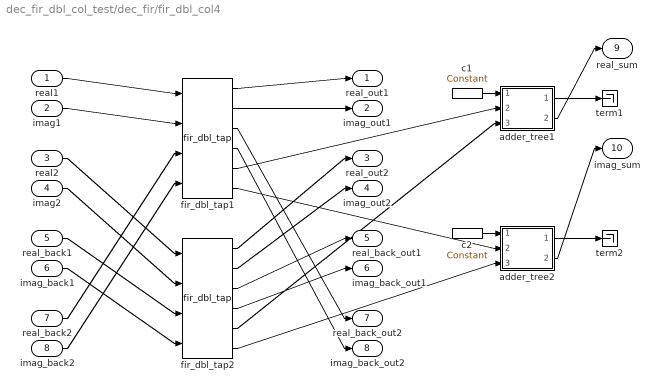
== system dec_fir_dbl_col_test/dec_fir/fir_dbl_col4 ==
  real1 : Inport
  imag1 : Inport  Port=2
  real2 : Inport  Port=3
  imag2 : Inport  Port=4
  real_back1 : Inport  Port=5
  imag_back1 : Inport  Port=6
  real_back2 : Inport  Port=7
  imag_back2 : Inport  Port=8
  adder_tree1 : Subsystem  AncestorBlock=casper_library_misc/adder_tree  mask(adder_tree){n_inputs=2, latency=2, adder_imp=DSP48, first_stage_hdl=off}
      mask prompts: n_inputs "Number of Inputs"; latency "Add Latency"; adder_imp "Adder implementation"; first_stage_hdl "Use behavioural HDL for first stage of adders"
      mask help:
      | Sums all inputs using a tree of adds and delays.
      |
      | Number of inputs: The number of inputs to the block to be summed
      | Add latency: The number of clock cycles to perform one addition (affects timing)..
      | Adder implementation: choice of fabric or DSP48E core, or behavioral HDL
      | Use behavioural HDL for first stage of adders: Causes the first stage of adders to be absorbed into DSP blocks if multipliers precede them (Virtex 5). Overrides Adder implementation
      mask init:
      | adder_tree_init(gcb, ...
      |     'n_inputs', n_inputs, ...
      |     'latency', latency, ...
      |     'adder_imp', adder_imp, ...
      |     'first_stage_hdl', first_stage_hdl);
      settings: AttributesFormatString=latency 2
      mask Help: eval('xlWeb(''http://casper.berkeley.edu/wiki/Adder_tree'')')
      mask StyleString: edit,edit,popup(Behavioral|Fabric|DSP48),checkbox
  adder_tree2 : Subsystem  AncestorBlock=casper_library_misc/adder_tree  mask(adder_tree){n_inputs=2, latency=2, adder_imp=DSP48, first_stage_hdl=off}
      mask prompts: n_inputs "Number of Inputs"; latency "Add Latency"; adder_imp "Adder implementation"; first_stage_hdl "Use behavioural HDL for first stage of adders"
      mask help:
      | Sums all inputs using a tree of adds and delays.
      |
      | Number of inputs: The number of inputs to the block to be summed
      | Add latency: The number of clock cycles to perform one addition (affects timing)..
      | Adder implementation: choice of fabric or DSP48E core, or behavioral HDL
      | Use behavioural HDL for first stage of adders: Causes the first stage of adders to be absorbed into DSP blocks if multipliers precede them (Virtex 5). Overrides Adder implementation
      mask init:
      | adder_tree_init(gcb, ...
      |     'n_inputs', n_inputs, ...
      |     'latency', latency, ...
      |     'adder_imp', adder_imp, ...
      |     'first_stage_hdl', first_stage_hdl);
      settings: AttributesFormatString=latency 2
      mask Help: eval('xlWeb(''http://casper.berkeley.edu/wiki/Adder_tree'')')
      mask StyleString: edit,edit,popup(Behavioral|Fabric|DSP48),checkbox
  c1 : xbsIndex_r4/Constant  arith_type=Signed (2's comp)  const=1  n_bits=16  bin_pt=14  explicit_period=on  period=1  equ=P=C  opselect=C  inp2=PCIN>>17  opr=+  inp1=P  carry=CIN  dbl_ovrd=off  block_type=constant
      settings: block_version=11.4
  c2 : xbsIndex_r4/Constant  arith_type=Signed (2's comp)  const=1  n_bits=16  bin_pt=14  explicit_period=on  period=1  equ=P=C  opselect=C  inp2=PCIN>>17  opr=+  inp1=P  carry=CIN  dbl_ovrd=off  block_type=constant
      settings: block_version=11.4
  fir_dbl_tap1 : casper_library_downconverter/fir_dbl_tap  SystemSampleTime=-1  factor=0.8  add_latency=2  mult_latency=3  coeff_bit_width=18  coeff_bin_pt=17
  fir_dbl_tap2 : casper_library_downconverter/fir_dbl_tap  SystemSampleTime=-1  factor=0.7  add_latency=2  mult_latency=3  coeff_bit_width=18  coeff_bin_pt=17
  term1 : Terminator
  term2 : Terminator
  real_out1 : Outport
  imag_out1 : Outport  Port=2
  real_out2 : Outport  Port=3
  imag_out2 : Outport  Port=4
  real_back_out1 : Outport  Port=5
  imag_back_out1 : Outport  Port=6
  real_back_out2 : Outport  Port=7
  imag_back_out2 : Outport  Port=8
  real_sum : Outport  Port=9
  imag_sum : Outport  Port=10
  wires:
  adder_tree1/1(sync_out) -> term1/1
  adder_tree2/1(sync_out) -> term2/1
  c1/1 -> adder_tree1/1(sync)
  c2/1 -> adder_tree2/1(sync)
  adder_tree1/2(dout) -> real_sum/1
  adder_tree2/2(dout) -> imag_sum/1
  real1/1 -> fir_dbl_tap1/1
  imag1/1 -> fir_dbl_tap1/2
  real_back2/1 -> fir_dbl_tap1/3
  imag_back2/1 -> fir_dbl_tap1/4
  fir_dbl_tap1/1 -> real_out1/1
  fir_dbl_tap1/2 -> imag_out1/1
  fir_dbl_tap1/3 -> real_back_out2/1
  fir_dbl_tap1/4 -> imag_back_out2/1
  fir_dbl_tap1/5 -> adder_tree1/2(din1)
  fir_dbl_tap1/6 -> adder_tree2/2(din1)
  real2/1 -> fir_dbl_tap2/1
  imag2/1 -> fir_dbl_tap2/2
  real_back1/1 -> fir_dbl_tap2/3
  imag_back1/1 -> fir_dbl_tap2/4
  fir_dbl_tap2/1 -> real_out2/1
  fir_dbl_tap2/2 -> imag_out2/1
  fir_dbl_tap2/3 -> real_back_out1/1
  fir_dbl_tap2/4 -> imag_back_out1/1
  fir_dbl_tap2/5 -> adder_tree1/3(din2)
  fir_dbl_tap2/6 -> adder_tree2/3(din2)

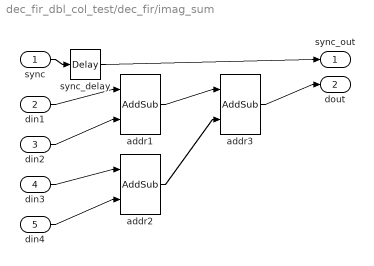
== system dec_fir_dbl_col_test/dec_fir/imag_sum ==
  sync : Inport
  din1 : Inport  Port=2
  din2 : Inport  Port=3
  din3 : Inport  Port=4
  din4 : Inport  Port=5
  addr1 : xbsIndex_r4/AddSub  mode=Addition  use_carryin=off  use_carryout=off  en=off  latency=2  precision=Full  arith_type=Unsigned  n_bits=16  bin_pt=14  quantization=Truncate  overflow=Wrap  dbl_ovrd=off  use_behavioral_HDL=off  hw_selection=DSP48  pipelined=on  use_rpm=on  block_type=addsub
  addr2 : xbsIndex_r4/AddSub  mode=Addition  use_carryin=off  use_carryout=off  en=off  latency=2  precision=Full  arith_type=Unsigned  n_bits=16  bin_pt=14  quantization=Truncate  overflow=Wrap  dbl_ovrd=off  use_behavioral_HDL=off  hw_selection=DSP48  pipelined=on  use_rpm=on  block_type=addsub
  addr3 : xbsIndex_r4/AddSub  mode=Addition  use_carryin=off  use_carryout=off  en=off  latency=2  precision=Full  arith_type=Unsigned  n_bits=16  bin_pt=14  quantization=Truncate  overflow=Wrap  dbl_ovrd=off  use_behavioral_HDL=off  hw_selection=DSP48  pipelined=on  use_rpm=on  block_type=addsub
  sync_delay : xbsIndex_r4/Delay  en=off  latency=4  dbl_ovrd=off  reg_retiming=on  block_type=delay
      settings: block_version=11.4
  sync_out : Outport
  dout : Outport  Port=2
  wires:
  sync/1 -> sync_delay/1
  sync_delay/1 -> sync_out/1
  din1/1 -> addr1/1
  din2/1 -> addr1/2
  din3/1 -> addr2/1
  din4/1 -> addr2/2
  addr1/1 -> addr3/1
  addr2/1 -> addr3/2
  addr3/1 -> dout/1

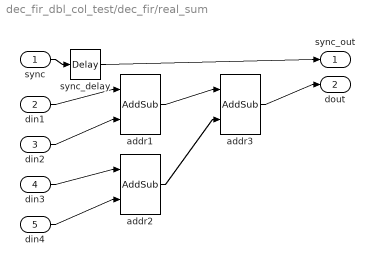
== system dec_fir_dbl_col_test/dec_fir/real_sum ==
  sync : Inport
  din1 : Inport  Port=2
  din2 : Inport  Port=3
  din3 : Inport  Port=4
  din4 : Inport  Port=5
  addr1 : xbsIndex_r4/AddSub  mode=Addition  use_carryin=off  use_carryout=off  en=off  latency=2  precision=Full  arith_type=Unsigned  n_bits=16  bin_pt=14  quantization=Truncate  overflow=Wrap  dbl_ovrd=off  use_behavioral_HDL=off  hw_selection=DSP48  pipelined=on  use_rpm=on  block_type=addsub
  addr2 : xbsIndex_r4/AddSub  mode=Addition  use_carryin=off  use_carryout=off  en=off  latency=2  precision=Full  arith_type=Unsigned  n_bits=16  bin_pt=14  quantization=Truncate  overflow=Wrap  dbl_ovrd=off  use_behavioral_HDL=off  hw_selection=DSP48  pipelined=on  use_rpm=on  block_type=addsub
  addr3 : xbsIndex_r4/AddSub  mode=Addition  use_carryin=off  use_carryout=off  en=off  latency=2  precision=Full  arith_type=Unsigned  n_bits=16  bin_pt=14  quantization=Truncate  overflow=Wrap  dbl_ovrd=off  use_behavioral_HDL=off  hw_selection=DSP48  pipelined=on  use_rpm=on  block_type=addsub
  sync_delay : xbsIndex_r4/Delay  en=off  latency=4  dbl_ovrd=off  reg_retiming=on  block_type=delay
      settings: block_version=11.4
  sync_out : Outport
  dout : Outport  Port=2
  wires:
  sync/1 -> sync_delay/1
  sync_delay/1 -> sync_out/1
  din1/1 -> addr1/1
  din2/1 -> addr1/2
  din3/1 -> addr2/1
  din4/1 -> addr2/2
  addr1/1 -> addr3/1
  addr2/1 -> addr3/2
  addr3/1 -> dout/1

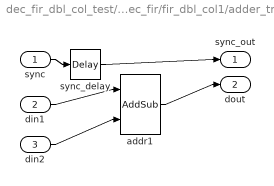
== system dec_fir_dbl_col_test/dec_fir/fir_dbl_col1/adder_tree1 ==
  sync : Inport
  din1 : Inport  Port=2
  din2 : Inport  Port=3
  addr1 : xbsIndex_r4/AddSub  mode=Addition  use_carryin=off  use_carryout=off  en=off  latency=2  precision=Full  arith_type=Unsigned  n_bits=16  bin_pt=14  quantization=Truncate  overflow=Wrap  dbl_ovrd=off  use_behavioral_HDL=off  hw_selection=DSP48  pipelined=on  use_rpm=on  block_type=addsub
  sync_delay : xbsIndex_r4/Delay  en=off  latency=2  dbl_ovrd=off  reg_retiming=on  block_type=delay
      settings: block_version=11.4
  sync_out : Outport
  dout : Outport  Port=2
  wires:
  sync/1 -> sync_delay/1
  sync_delay/1 -> sync_out/1
  din1/1 -> addr1/1
  din2/1 -> addr1/2
  addr1/1 -> dout/1

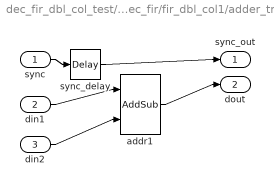
== system dec_fir_dbl_col_test/dec_fir/fir_dbl_col1/adder_tree2 ==
  sync : Inport
  din1 : Inport  Port=2
  din2 : Inport  Port=3
  addr1 : xbsIndex_r4/AddSub  mode=Addition  use_carryin=off  use_carryout=off  en=off  latency=2  precision=Full  arith_type=Unsigned  n_bits=16  bin_pt=14  quantization=Truncate  overflow=Wrap  dbl_ovrd=off  use_behavioral_HDL=off  hw_selection=DSP48  pipelined=on  use_rpm=on  block_type=addsub
  sync_delay : xbsIndex_r4/Delay  en=off  latency=2  dbl_ovrd=off  reg_retiming=on  block_type=delay
      settings: block_version=11.4
  sync_out : Outport
  dout : Outport  Port=2
  wires:
  sync/1 -> sync_delay/1
  sync_delay/1 -> sync_out/1
  din1/1 -> addr1/1
  din2/1 -> addr1/2
  addr1/1 -> dout/1

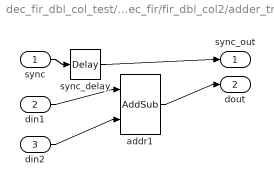
== system dec_fir_dbl_col_test/dec_fir/fir_dbl_col2/adder_tree1 ==
  sync : Inport
  din1 : Inport  Port=2
  din2 : Inport  Port=3
  addr1 : xbsIndex_r4/AddSub  mode=Addition  use_carryin=off  use_carryout=off  en=off  latency=2  precision=Full  arith_type=Unsigned  n_bits=16  bin_pt=14  quantization=Truncate  overflow=Wrap  dbl_ovrd=off  use_behavioral_HDL=off  hw_selection=DSP48  pipelined=on  use_rpm=on  block_type=addsub
  sync_delay : xbsIndex_r4/Delay  en=off  latency=2  dbl_ovrd=off  reg_retiming=on  block_type=delay
      settings: block_version=11.4
  sync_out : Outport
  dout : Outport  Port=2
  wires:
  sync/1 -> sync_delay/1
  sync_delay/1 -> sync_out/1
  din1/1 -> addr1/1
  din2/1 -> addr1/2
  addr1/1 -> dout/1

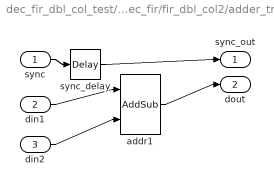
== system dec_fir_dbl_col_test/dec_fir/fir_dbl_col2/adder_tree2 ==
  sync : Inport
  din1 : Inport  Port=2
  din2 : Inport  Port=3
  addr1 : xbsIndex_r4/AddSub  mode=Addition  use_carryin=off  use_carryout=off  en=off  latency=2  precision=Full  arith_type=Unsigned  n_bits=16  bin_pt=14  quantization=Truncate  overflow=Wrap  dbl_ovrd=off  use_behavioral_HDL=off  hw_selection=DSP48  pipelined=on  use_rpm=on  block_type=addsub
  sync_delay : xbsIndex_r4/Delay  en=off  latency=2  dbl_ovrd=off  reg_retiming=on  block_type=delay
      settings: block_version=11.4
  sync_out : Outport
  dout : Outport  Port=2
  wires:
  sync/1 -> sync_delay/1
  sync_delay/1 -> sync_out/1
  din1/1 -> addr1/1
  din2/1 -> addr1/2
  addr1/1 -> dout/1

== system dec_fir_dbl_col_test/dec_fir/fir_dbl_col3/adder_tree1 ==
  sync : Inport
  din1 : Inport  Port=2
  din2 : Inport  Port=3
  addr1 : xbsIndex_r4/AddSub  mode=Addition  use_carryin=off  use_carryout=off  en=off  latency=2  precision=Full  arith_type=Unsigned  n_bits=16  bin_pt=14  quantization=Truncate  overflow=Wrap  dbl_ovrd=off  use_behavioral_HDL=off  hw_selection=DSP48  pipelined=on  use_rpm=on  block_type=addsub
  sync_delay : xbsIndex_r4/Delay  en=off  latency=2  dbl_ovrd=off  reg_retiming=on  block_type=delay
      settings: block_version=11.4
  sync_out : Outport
  dout : Outport  Port=2
  wires:
  sync/1 -> sync_delay/1
  sync_delay/1 -> sync_out/1
  din1/1 -> addr1/1
  din2/1 -> addr1/2
  addr1/1 -> dout/1

== system dec_fir_dbl_col_test/dec_fir/fir_dbl_col3/adder_tree2 ==
  sync : Inport
  din1 : Inport  Port=2
  din2 : Inport  Port=3
  addr1 : xbsIndex_r4/AddSub  mode=Addition  use_carryin=off  use_carryout=off  en=off  latency=2  precision=Full  arith_type=Unsigned  n_bits=16  bin_pt=14  quantization=Truncate  overflow=Wrap  dbl_ovrd=off  use_behavioral_HDL=off  hw_selection=DSP48  pipelined=on  use_rpm=on  block_type=addsub
  sync_delay : xbsIndex_r4/Delay  en=off  latency=2  dbl_ovrd=off  reg_retiming=on  block_type=delay
      settings: block_version=11.4
  sync_out : Outport
  dout : Outport  Port=2
  wires:
  sync/1 -> sync_delay/1
  sync_delay/1 -> sync_out/1
  din1/1 -> addr1/1
  din2/1 -> addr1/2
  addr1/1 -> dout/1

== system dec_fir_dbl_col_test/dec_fir/fir_dbl_col4/adder_tree1 ==
  sync : Inport
  din1 : Inport  Port=2
  din2 : Inport  Port=3
  addr1 : xbsIndex_r4/AddSub  mode=Addition  use_carryin=off  use_carryout=off  en=off  latency=2  precision=Full  arith_type=Unsigned  n_bits=16  bin_pt=14  quantization=Truncate  overflow=Wrap  dbl_ovrd=off  use_behavioral_HDL=off  hw_selection=DSP48  pipelined=on  use_rpm=on  block_type=addsub
  sync_delay : xbsIndex_r4/Delay  en=off  latency=2  dbl_ovrd=off  reg_retiming=on  block_type=delay
      settings: block_version=11.4
  sync_out : Outport
  dout : Outport  Port=2
  wires:
  sync/1 -> sync_delay/1
  sync_delay/1 -> sync_out/1
  din1/1 -> addr1/1
  din2/1 -> addr1/2
  addr1/1 -> dout/1

== system dec_fir_dbl_col_test/dec_fir/fir_dbl_col4/adder_tree2 ==
  sync : Inport
  din1 : Inport  Port=2
  din2 : Inport  Port=3
  addr1 : xbsIndex_r4/AddSub  mode=Addition  use_carryin=off  use_carryout=off  en=off  latency=2  precision=Full  arith_type=Unsigned  n_bits=16  bin_pt=14  quantization=Truncate  overflow=Wrap  dbl_ovrd=off  use_behavioral_HDL=off  hw_selection=DSP48  pipelined=on  use_rpm=on  block_type=addsub
  sync_delay : xbsIndex_r4/Delay  en=off  latency=2  dbl_ovrd=off  reg_retiming=on  block_type=delay
      settings: block_version=11.4
  sync_out : Outport
  dout : Outport  Port=2
  wires:
  sync/1 -> sync_delay/1
  sync_delay/1 -> sync_out/1
  din1/1 -> addr1/1
  din2/1 -> addr1/2
  addr1/1 -> dout/1
